simulink model "CNC_MPC"  (R2024b)
settings: Solver=ode1  StartTime=0.0  StopTime=10  FixedStep=0.002  RelTol=1e-3  EnableMultiTasking=on
PostLoadFcn:
  | qc_set_target_type(getConfigSet(bdroot, 'QUARC config'));
  | addpath(fileparts(fileparts(get_param(bdroot,'FileName'))));
StartFcn:
  | addpath(fullfile(fileparts(get_param(bdroot,'FileName')),'..','scripts'));
  | run_and_save_deferred(bdroot, 'start');
StopFcn:
  | addpath(fullfile(fileparts(get_param(bdroot,'FileName')),'..','scripts'));
  | run_and_save_deferred(bdroot, 'stop');
undefined symbols (not defined in the file): Aa, Ba, Ca, Dm, Eyflat, Fq, Gq, HIL, L, N, qc_get_step_size, qp_iter, Qref, REF_p, REF_q, Ts, umax, w, x0
libraries: quarc_library x4
settings Model: SimulationMode=external  Creator=Giuliano Livi  LastModifiedBy=Giuliano Livi
settings SolverCC: AlgebraicLoopSolver=TrustRegion  PositivePriorityOrder=on
settings DataIOCC: LimitDataPoints=on  SaveFormat=Array  SignalLoggingSaveFormat=ModelDataLogs
settings OptimizationCC: ExpressionDepthLimit=2147483647  InitFltsAndDblsToZero=on
settings DebuggingCC: SaveWithParameterizedLinksMsg=none  UnderspecifiedInitializationDetection=Classic  MergeDetectMultiDrivingBlocksExec=none  SolverPrmCheckMsg=warning  MultiTaskDSMMsg=warning  MultiTaskCondExecSysMsg=none  FcnCallInpInsideContextMsg=warning  UnconnectedInputMsg=warning  UnconnectedOutputMsg=warning  UnconnectedLineMsg=warning  StateNameClashWarn=warning  SFUnexpectedBacktrackingDiag=warning  SFNoUnconditionalDefaultTransitionDiag=warning  SFExecutionAtInitializationDiag=none  ArithmeticOperatorsInVariantConditions=warning
settings ModelReferenceCC: EnableRefExpFcnMdlSchedulingChecks=on  PropagateSignalLabelsOutOfModel=off
settings SFSimCC: SimUseLocalCustomCode=off  CustomCodeUndefinedFunction=UseInterfaceOnly
settings RTWCC: Description=QUARC Win64 Target Using Toolchain  SystemTargetFile=quarc_win64.tlc  TemplateMakefile=quarc_default_tmf  RTWUseLocalCustomCode=off  Toolchain=QUARC win64 | nmake (64-bit Windows)  BuildConfiguration=Faster Runs  GPUComputeCapability=3.5
settings CodeAppCC: StateflowObjectComments=on
settings STFCustomTargetCC: ConcurrentExecutionCompliant=on  GRTInterface=on  UseToolchainInfoCompliant=on  SystemTargetFile=quarc_win64.tlc
settings GRTTargetCC: TargetLangStandard=C89/C90 (ANSI)  ParMdlRefBuildCompliant=off  CompOptLevelCompliant=off  CombineOutputUpdateFcns=off  MatFileLogging=off  CPPClassGenCompliant=off  GRTInterface=on  ExtMode=on  ExtModeMexFile=quarc_comm
settings ConfigComp: CovMetricSettings=dw  CovSaveCumulativeToWorkspaceVar=on  CovSaveSingleToWorkspaceVar=on  CovExternalEMLEnable=off

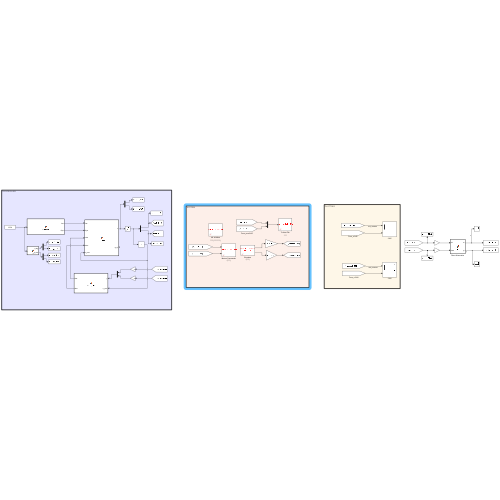
[thumbnail: Simulink's stored preview of the top-level diagram]
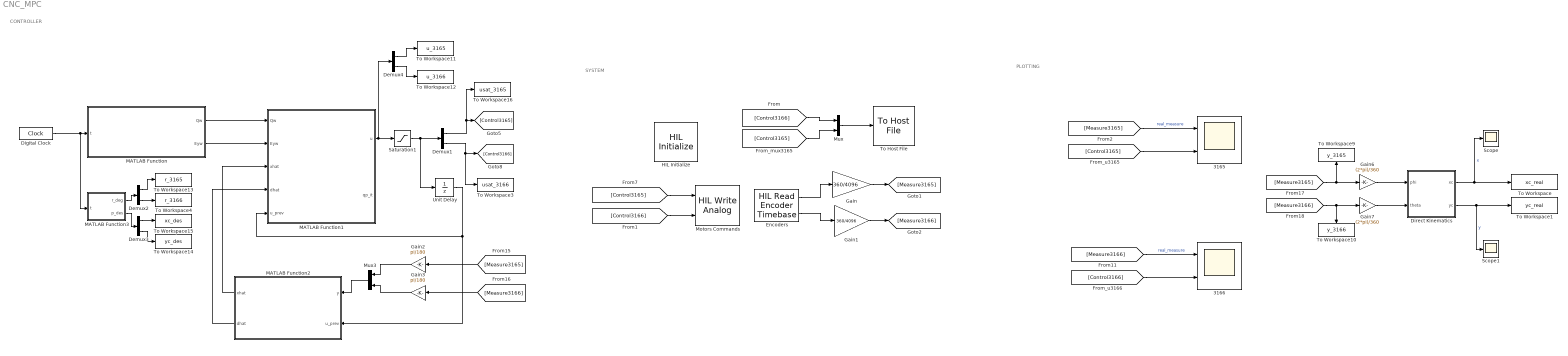
== system CNC_MPC ==
  note: PLOTTING
  note: SYSTEM
  note: CONTROLLER
  3165 : Scope  NumInputPorts=2
  3166 : Scope  NumInputPorts=2
  Demux{1..4} (4 alike) : Demux  Outputs=2
  Digital Clock : DigitalClock  SampleTime=Ts
  Direct Kinematics : MATLAB Function  TreatAsAtomicUnit=on  SystemSampleTime=0.002
  Encoders : quarc_library/Data Acquisition/Generic/Timebases/HIL Read Encoder Timebase  object_name=HIL-1  clock=0  channels=0:1  active=on  vector_output=off  data_type_mode=Inherit via back propagation  data_type=double  overflow_mode=Error on overflow  samples_in_buffer=max(ceil(1/qc_get_step_size), 1)
  Gain : Gain  Gain=360/4096
  Gain1 : Gain  Gain=360/4096
  Gain2 : Gain  Gain=pi/180
  Gain3 : Gain  Gain=pi/180
  Gain6 : Gain  Gain=(2*pi)/360
  Gain7 : Gain  Gain=(2*pi)/360
  HIL Initialize : quarc_library/Data Acquisition/Generic/Configuration/HIL Initialize  object_name=HIL-1  board_type=q2_usb  board_number=0  board_options=d0=digital;d1=digital;led=auto;update_rate=normal;decimation=1  exclusive=off  active=off  hardware_clocks=[0]  clock_modes=[]  initial_clock_frequencies=[]  set_clock_params_at_start=off  set_clock_params_at_switch_in=off  set_clock_frequencies_at_start=off  set_clock_frequencies_at_switch_in=off  analog_input_channels=[0:1]  analog_input_configurations=[]  analog_input_maximums=10  analog_input_minimums=-10  set_analog_input_params_at_start=on  set_analog_input_params_at_switch_in=off  analog_output_channels=[0:1]  analog_output_maximums=10  analog_output_minimums=-10  initial_analog_outputs=[0]  final_analog_outputs=[0]  watchdog_analog_outputs=0  set_analog_output_params_at_start=on  set_analog_output_params_at_switch_in=off  set_analog_outputs_at_start=on  set_analog_outputs_at_switch_in=off  set_analog_outputs_at_terminate=on  set_analog_outputs_at_switch_out=off  set_analog_outputs_on_watchdog=off  digital_input_channels=[]  digital_output_channels=[]  digital_output_configuration=[]  initial_digital_outputs=[1]  final_digital_outputs=[1]  watchdog_digital_outputs=[1]  set_digital_output_params_at_start=off  set_digital_output_params_at_switch_in=off  set_digital_outputs_at_start=on  set_digital_outputs_at_switch_in=off  set_digital_outputs_at_terminate=on  set_digital_outputs_at_switch_out=off  set_digital_outputs_on_watchdog=off  encoder_channels=[0:1]  quadrature=[4]  encoder_filter_frequency=[]  initial_encoder_counts=[0]  set_encoder_params_at_start=on  set_encoder_params_at_switch_in=off  set_encoder_counts_at_start=on  set_encoder_counts_at_switch_in=off  pwm_channels=[]  pwm_modes=[0]  pwm_frequency=1/0.020  pwm_configuration=[]  pwm_alignment=[]  pwm_polarity=[]  pwm_leading_deadband=[]  pwm_trailing_deadband=[]  initial_pwm_outputs=[0]  final_pwm_outputs=[0]  watchdog_pwm_outputs=[0]  set_pwm_params_at_start=on  set_pwm_params_at_switch_in=off  set_pwm_outputs_at_start=on  set_pwm_outputs_at_switch_in=off  set_pwm_outputs_at_terminate=on  set_pwm_outputs_at_switch_out=off  set_pwm_outputs_on_watchdog=off  other_output_channels=[]  initial_other_outputs=[]  final_other_outputs=[]  watchdog_other_outputs=[]  set_other_outputs_at_start=off  set_other_outputs_at_switch_in=off  set_other_outputs_at_terminate=off  set_other_outputs_at_switch_out=off  set_other_outputs_on_watchdog=off
  MATLAB Function : MATLAB Function  TreatAsAtomicUnit=on
  MATLAB Function1 : MATLAB Function  TreatAsAtomicUnit=on
  MATLAB Function2 : MATLAB Function  TreatAsAtomicUnit=on
  MATLAB Function3 : MATLAB Function  TreatAsAtomicUnit=on
  Motors Commands : quarc_library/Data Acquisition/Generic/Immediate I//O/HIL Write Analog  object_name=HIL-1  channels=0:1  sample_time=-1  active=off  vector_input=off
  Mux : Mux  Inputs=2
  Mux3 : Mux  Inputs=2
  Saturation1 : Saturate  UpperLimit=6  LowerLimit=-6
  Scope : Scope
  Scope1 : Scope
  To Host File : quarc_library/Sinks/To Host/To Host File  source=Specify via dialog (do not evaluate)  file_name=data_%{date}_%{time}.mat  variable_name=data  decimation=1  sample_time=-1  file_format=MAT-file v.4  options=No header or footer  append=off  final_file_name=data_09-Nov-2026_17-49-36.mat  encoding=Default  bitrate=2000000
  To Workspace : ToWorkspace  VariableName=xc_real  SaveFormat=Structure With Time  SampleTime=-1
  To Workspace1 : ToWorkspace  VariableName=yc_real  SaveFormat=Structure With Time  SampleTime=-1
  To Workspace10 : ToWorkspace  VariableName=y_3166  SaveFormat=Structure With Time  SampleTime=0.002
  To Workspace11 : ToWorkspace  VariableName=u_3165  SaveFormat=Timeseries  SampleTime=0.002
  To Workspace12 : ToWorkspace  VariableName=u_3166  SaveFormat=Timeseries  SampleTime=0.002
  To Workspace13 : ToWorkspace  VariableName=r_3165  SaveFormat=Timeseries  SampleTime=0.002
  To Workspace14 : ToWorkspace  VariableName=yc_des  SaveFormat=Timeseries  SampleTime=0.002
  To Workspace15 : ToWorkspace  VariableName=xc_des  SaveFormat=Timeseries  SampleTime=0.002
  To Workspace16 : ToWorkspace  VariableName=usat_3165  SaveFormat=Timeseries  SampleTime=0.002
  To Workspace3 : ToWorkspace  VariableName=usat_3166  SaveFormat=Timeseries  SampleTime=0.002
  To Workspace4 : ToWorkspace  VariableName=r_3166  SaveFormat=Timeseries  SampleTime=0.002
  To Workspace9 : ToWorkspace  VariableName=y_3165  SaveFormat=Structure With Time  SampleTime=0.002
  Unit Delay : UnitDelay  SampleTime=Ts  HasFrameUpgradeWarning=on
  wires:
  [Measure3166] -> 3166/1  "real_measure"
  Gain7/1 -> Direct Kinematics/2(theta)
  Gain6/1 -> Direct Kinematics/1(phi)
  Mux/1 -> To Host File/1
  [Measure3166] -> To Workspace10/1, Gain7/1
  [Control3166] -> Motors Commands/2
  Gain1/1 -> [Measure3166]
  Gain/1 -> [Measure3165]
  Direct Kinematics/1(xc) -> To Workspace/1, Scope/1  "x"
  [Measure3165] -> 3165/1  "real_measure"
  [Measure3165] -> Gain6/1, To Workspace9/1
  Direct Kinematics/2(yc) -> Scope1/1, To Workspace1/1  "y"
  Encoders/2 -> Gain1/1
  Encoders/1 -> Gain/1
  [Control3166] -> Mux/1
  [Control3165] -> Motors Commands/1
  MATLAB Function3/1(r_deg) -> Demux2/1
  Demux2/1 -> To Workspace13/1
  MATLAB Function3/2(p_des) -> Demux3/1
  Demux4/2 -> To Workspace12/1
  Demux3/2 -> To Workspace14/1
  Unit Delay/1 -> MATLAB Function2/2(u_prev), MATLAB Function1/5(u_prev)
  Demux4/1 -> To Workspace11/1
  [Measure3166] -> Gain3/1
  Demux3/1 -> To Workspace15/1
  Mux3/1 -> MATLAB Function2/1(y)
  MATLAB Function1/1(u) -> Saturation1/1, Demux4/1
  Demux1/2 -> To Workspace3/1, [Control3166]
  MATLAB Function2/1(xhat) -> MATLAB Function1/3(xhat)
  MATLAB Function/1(Qw) -> MATLAB Function1/1(Qw)
  Digital Clock/1 -> MATLAB Function3/1(t), MATLAB Function/1(t)
  Demux1/1 -> To Workspace16/1, [Control3165]
  MATLAB Function2/2(dhat) -> MATLAB Function1/4(dhat)
  Saturation1/1 -> Unit Delay/1, Demux1/1
  MATLAB Function/2(Eyw) -> MATLAB Function1/2(Eyw)
  [Measure3165] -> Gain2/1
  Demux2/2 -> To Workspace4/1
  Gain2/1 -> Mux3/1
  Gain3/1 -> Mux3/2
  [Control3165] -> 3165/2
  [Control3166] -> 3166/2
  [Control3165] -> Mux/2

== matlab function CNC_MPC/Direct Kinematics ==
  data: phi input; xc output; theta input; yc output
function [xc, yc] = fcn(phi, theta)
l = 0.127;
a = 2 - sin(theta) - cos(phi);
b = cos(theta) - sin(phi);
s = sqrt(a^2 + b^2);
h = l*sqrt(1 - s^2/4);

% Nonlinear forward kinematics of point C
xc = l/2*(2 - sin(theta) + cos(phi)) - h*b/s;
yc = l/2*(cos(theta) + sin(phi))     + h*a/s;

== matlab function CNC_MPC/MATLAB Function ==
  data: t input; Qw output; Eyw output; Qref parameter; Eyflat parameter; N parameter; Ts parameter
function [Qw, Eyw] = refWindow(t, Qref, Eyflat, N, Ts)
%#codegen
% MATLAB Function block: preview window r_{k+1} ... r_{k+N} for the MPC.
%   k      : current sample index, 0-based (input port, e.g. from a counter)
%   Qref   = REF_q   [2 x n]  joint reference [rad]
%   Eyflat = REF_Ey  [4 x n]  contour/lag maps Ey = [n'; t']*J, column-major
%   N      = mpc horizon
%   (Qref, Eyflat, N: declare them as PARAMETERS in the Ports and Data Manager)
% Outputs, one column per horizon step j = 1..N:
%   Qw [2xN] joint reference,  Eyw [4xN] (reshape column j to 2x2 to get Ey_{k+j})
k   = round(t/Ts);                 % sample index (0-based) from the time
nS  = size(Qref, 2);
idx = min(k + (2:N+1), nS);
Qw  = Qref(:, idx);
Eyw = Eyflat(:, idx);
end

== matlab function CNC_MPC/MATLAB Function1 ==
  data: Qw input; Eyw input; xhat input; u output; dhat input; u_prev input; qp_it output; Fq parameter; Gq parameter; umax parameter; Dm parameter; E0 parameter; qp_iter parameter; w parameter
function [u, qp_it] = mpc_step(Qw, Eyw, xhat, dhat, u_prev, Fq, Gq, umax, Dm, E0, qp_iter, w)
%#codegen
% MATLAB Function block: LTV MPC on contour / lag error, one QP per sample.
% Inputs (signals):
%   xhat   [4x1]  state estimate [phi; dphi; theta; dtheta]        (kalman_step)
%   dhat   [2x1]  input-disturbance estimate [V]                   (kalman_step)
%   Qw     [2xN]  window of q_ref,{k+j} [rad]                         (refWindow)
%   Eyw    [4xN]  window of Ey_{k+j} = [n'; t'] * J  (column-major)  (refWindow)
%   u_prev [2x1]  input applied at the previous sample [V]  (after saturation, Unit Delay)
% Parameters: Fq = mpc.Fq, Gq = mpc.Gq, Dm = mpc.Dm, E0 = mpc.E0, w = mpc.w (struct),
%             umax = mpc.umax, qp_iter = mpc.qp_iter
% Outputs: u [2x1] voltage to apply [V],  qp_it = active-set iterations used
%
% Decision variable V = U + d (the plant sees u + d):  q_pred = Fq*x + Gq*V
%   cost = sum_j [ qc*e_c,j^2 + ql*e_l,j^2 ] + r*|dU|^2
%   e_j = Ey_j * (q_j - q_ref,j),    dU = Dm*V - E0*(u_prev + d)
%   -umax <= u = V - d <= umax   ->   d - umax <= V <= d + umax
 
% Everything is prepared for the solver:

N  = size(Eyw, 2);
nV = size(Gq, 2);
x  = xhat(:);  
d = dhat(:);
 
% 1. Linearized contour/lag error along the horizon:  e = M*V + c
M = zeros(2*N, nV);
c = zeros(2*N, 1);
for j = 1:N
    r2 = 2*j-1:2*j;
    Ej = reshape(Eyw(:,j), 2, 2);
    M(r2, :) = Ej*Gq(r2, :);
    c(r2) = Ej*(Fq(r2,:)*x - Qw(:,j));          % e = Ey*(q_pred - q_ref)
end
Wv = repmat([w.qc; w.ql], N, 1);
 
% 2. QP:  min 0.5*V'*H*V + f'*V   s.t.  lb <= V <= ub
H = 2*(M'*(Wv.*M) + w.r*(Dm'*Dm));
f = 2*(M'*(Wv.*c) - w.r*(Dm'*(E0*(u_prev(:) + d))));
H = 0.5*(H + H');                                  % exact symmetry
lb = repmat(d - umax, nV/2, 1);
ub = repmat(d + umax, nV/2, 1);
 
[V, qp_it] = box_qp(H, f, lb, ub, qp_iter);
 
% 3. Receding horizon: apply only the first move
u = V(1:2) - d;
end
 
%% ------------------------------------------------------------------------
function [U, it] = box_qp(H, f, lb, ub, maxit)
% Exact solver for a small QP with box constraints (primal-dual active set).
% Starts from the unconstrained optimum: if it is feasible (no saturation),
% the answer is exact after one linear solve.
n  = numel(f);
U  = -(H\f);
it = 0;
lo = U < lb;
up = U > ub;
while (any(lo) || any(up)) && it < maxit
    it = it + 1;
    % Solve with the active variables fixed at their bound
    Hm = H;  rhs = -f;
    for i = 1:n
        if lo(i) || up(i)
            Hm(i, :) = 0;  Hm(i, i) = 1;
            if lo(i), rhs(i) = lb(i); else, rhs(i) = ub(i); end
        end
    end
    U = Hm\rhs;
    g = H*U + f;                                   % gradient = minus the multipliers
    % Keep a bound only if the gradient pushes outwards, add the violated ones
    lo_new = (U < lb - 1e-12) | (lo & g > 0);
    up_new = (U > ub + 1e-12) | (up & g < 0);
    if isequal(lo_new, lo) && isequal(up_new, up)
        break;                                     % KKT conditions satisfied
    end
    lo = lo_new;  up = up_new;
end
U = min(max(U, lb), ub);                           % safety clip
end

== matlab function CNC_MPC/MATLAB Function2 ==
  data: y input; xhat output; u_prev input; dhat output; Aa parameter; Ba parameter; Ca parameter; x0 parameter; L parameter
function [xhat, dhat] = kalman_step(y, u_prev, Aa, Ba, Ca, x0, L)
%#codegen
% MATLAB Function block: steady-state Kalman filter with input-disturbance states.
%   y      [2x1] measured joint angles [rad]  (encoder deg * pi/180)
%   u_prev [2x1] input APPLIED at the previous sample [V] (after the saturation, Unit Delay)
%   Aa, Ba, Ca, L, x0 : PARAMETERS  (est.Aa, est.Ba, est.Ca, est.L, initial state [6x1])
% Outputs (estimate at time k, after using y_k):
%   xhat [4x1] = [phi; dphi; theta; dtheta]     dhat [2x1] input disturbance [V]
% Model: xa = [x; d], x_{k+1} = A x + B (u + d), d_{k+1} = d, y = [phi; theta]
 
persistent xa
if isempty(xa)
    xa = x0;                       % start: robot at home, at rest, no disturbance
else
    xa = Aa*xa + Ba*u_prev;        % time update with the input actually applied at k-1
end
xa = xa + L*(y - Ca*xa);           % measurement update with y_k
 
xhat = xa(1:4);
dhat = xa(5:6);
end

== matlab function CNC_MPC/MATLAB Function3 ==
  data: t input; r_deg output; p_des output; REF_q parameter; REF_p parameter; Ts parameter
function [r_deg, p_des] = fcn(t, REF_q, REF_p, Ts)
i = min(round(t/Ts) + 1, size(REF_q, 2));   % current sample (MATLAB index)
r_deg = REF_q(:, i) * 180/pi;               % encoder degrees
p_des = REF_p(:, i);                        % [x; y] desired [m]
end
